simulink model "demoS175WindCurrentAutopilot"  (R2022a)
settings: Solver=ode45  StartTime=0.0  StopTime=500  FixedStep=Auto  RelTol=1e-10  EnableMultiTasking=on
PreLoadFcn:
  | TT=50;
InitFcn:
  | dataContainer;
StopFcn:
  | shipsOrient;
undefined symbols (not defined in the file): aH, AR, B, cpr, cpv, cRr, cRrrr, cRrrv, cRX, D, Delta, detM, epsilon, g, ga, GM, kk, Kp, Kphi, Kr, Krphiphi, Krrphi, Krrr, Kv, Kvphiphi, Kvrr, Kvvphi, Kvvr, Kvvv, L, lx, m, m11, m22, m32, m33, m42, m44, magnitude, mx, my, nabla, Np, Nphi, Nr, Nrphiphi, Nrrphi, Nrrr, Nv, Nvphiphi, Nvrr, Nvvphi, Nvvr, Nvvv, rho, tau, wp, xH, xp, Xphiphi ... (+18)
libraries: simulink_extras x8, mssSimulink x5, simulink x4
settings Model: Creator=AP  LastModifiedBy=thor
settings SolverCC: AlgebraicLoopSolver=TrustRegion
settings DataIOCC: LimitDataPoints=on  SaveFormat=Array  SignalLoggingSaveFormat=ModelDataLogs  ReturnWorkspaceOutputs=off
settings OptimizationCC: ExpressionDepthLimit=2147483647  InitFltsAndDblsToZero=on  LifeSpan=inf
settings DebuggingCC: SaveWithParameterizedLinksMsg=none  UnderspecifiedInitializationDetection=Classic  MergeDetectMultiDrivingBlocksExec=none  SignalResolutionControl=TryResolveAllWithWarning  SolverPrmCheckMsg=warning  MultiTaskDSMMsg=warning  MultiTaskCondExecSysMsg=none  FcnCallInpInsideContextMsg=warning  UnconnectedInputMsg=warning  UnconnectedOutputMsg=warning  UnconnectedLineMsg=warning  StateNameClashWarn=warning  SFUnexpectedBacktrackingDiag=warning  SFNoUnconditionalDefaultTransitionDiag=warning  SFExecutionAtInitializationDiag=none  SFMachineParentedDataDiag=warning  ArithmeticOperatorsInVariantConditions=warning
settings HardwareCC: ProdBitPerPointer=32  ProdBitPerSizeT=32  ProdBitPerPtrDiffT=32  ProdLargestAtomicFloat=None  ProdIntDivRoundTo=Undefined  ProdEndianess=Unspecified  ProdWordSize=32  ProdHWDeviceType=32-bit Generic
settings ModelReferenceCC: PropagateSignalLabelsOutOfModel=off
settings SFSimCC: SimUseLocalCustomCode=off  CustomCodeUndefinedFunction=UseInterfaceOnly
settings RTWCC: RTWUseLocalCustomCode=off  DLArmComputeVersion=19.05
settings CodeAppCC: StateflowObjectComments=on
settings GRTTargetCC: TargetFcnLib=ansi_tfl_tmw.mat  TargetLangStandard=C89/C90 (ANSI)  CombineOutputUpdateFcns=off  GRTInterface=on
settings ConfigComp: CovMetricSettings=dw  CovSaveCumulativeToWorkspaceVar=on  CovSaveSingleToWorkspaceVar=on  CovExternalEMLEnable=off

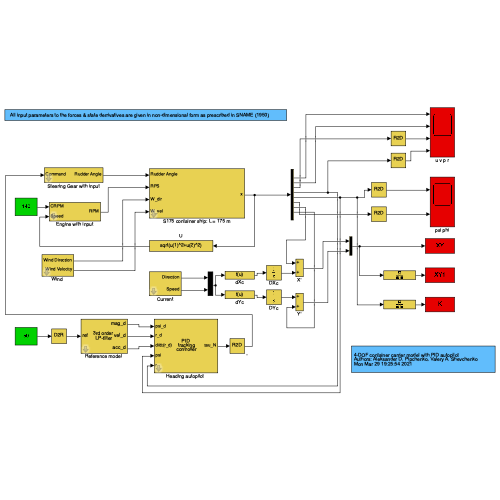
[thumbnail: Simulink's stored preview of the top-level diagram]
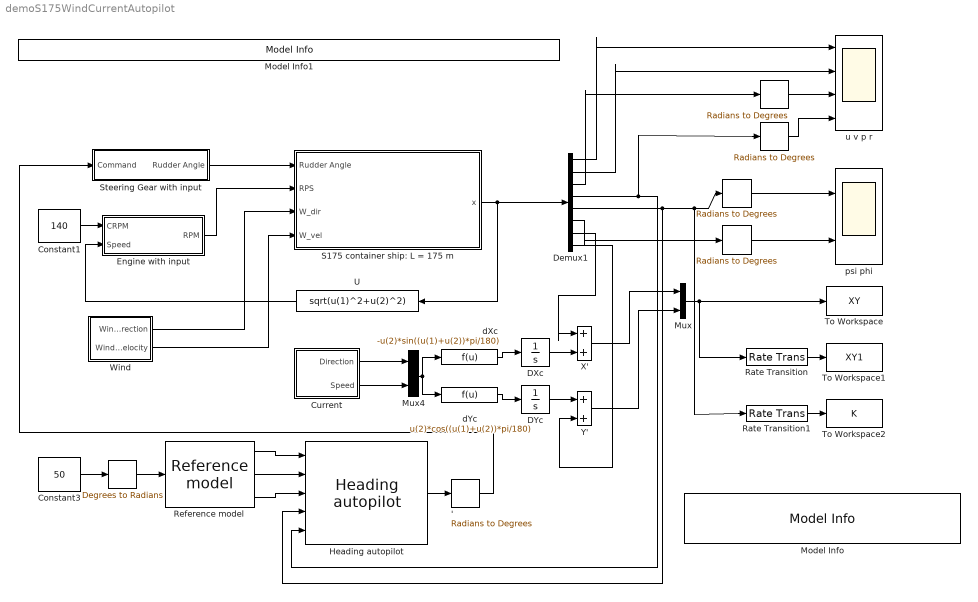
== system demoS175WindCurrentAutopilot ==
  "   " : simulink_extras/Transformations/Radians to Degrees
  "    " : simulink_extras/Transformations/Radians to Degrees
  "     " : simulink_extras/Transformations/Degrees to Radians
  "      " : simulink_extras/Transformations/Radians to Degrees
  "                " : simulink_extras/Transformations/Radians to Degrees
  "               '" : simulink_extras/Transformations/Radians to Degrees
  Constant1 : Constant  Value=140
  Constant3 : Constant  Value=50
  Current : Subsystem  AncestorBlock=Maneuvering/Environment/Current  mask(Environment disturbance/ Sea Current){CD=5, CS=2}
      mask prompts: CD "Current Direction, deg"; CS "Current Speed, knots"
      mask help: Apply current speed and direction to appropriate gaps
  DXc : Integrator
  DYc : Integrator
  Demux1 : Demux  Outputs=8
  Engine with input : Subsystem  mask(Engine (simplified)){IRPM=140, MaxRPM=160, MinRPM=0, T_rpm=5.65, RevV=0, RTH=0, OTE=Revs per second}
      mask prompts: IRPM "Initial RPM, revs/min"; MaxRPM "Maximum RPM"; MinRPM "Minimum RPM"; T_rpm "Derrivative Time Constant"; RevV "Reversal speed, m/s"; RTH "RPM to keep ahead at crash stop, revs/min"; OTE "Output time expression"
      mask help:
      | Insert the reversal speed, and RPM ahead you want to hold
      | while ship not reach this speed at crash stop maneuver
      mask init:
      | if OTE=='Revs per minute'
      | 	TEX = 1;
      | elseif OTE=='Revs per second'
      | 	TEX = 1/60;
      | end;
      mask TypeOptions OTE: Revs per minute | Revs per second
  "Heading autopilot " : mssSimulink/Control/Autopilots/Heading autopilot  T_nomoto=107.3  K_nomoto=0.185  Kp=2  Td=50  Ti=100
  Model Info : simulink/Model-Wide Utilities/Model Info  Frame=on  DisplayStringWithTags=|  HorizontalTextAlignment=Left  LeftAlignmentValue=0.02
      | 4-DOF container carrier model with PID autopilot
      | Authors: Aleksander D. Pipchenko, Valery A. Shevchenko
      | %<LastModificationDate>
  Model Info1 : simulink/Model-Wide Utilities/Model Info  Frame=on  DisplayStringWithTags=All input parameters to the forces & state derrivatives are given in non-dimensional form as prescribed in SNAME (1950)  HorizontalTextAlignment=Left  LeftAlignmentValue=0.02
  Mux : Mux  Inputs=2
  Mux4 : Mux  Inputs=2
  Rate Transition : RateTransition  OutPortSampleTime=TT
  Rate Transition1 : RateTransition  OutPortSampleTime=TT
  "Reference model " : mssSimulink/Guidance/Reference model  v_max=1.0  zeta_d=1.0  w_d=0.1
  S175 container ship: L = 175 m : Subsystem  mask(Container ship 4-DOF model / Simulink based){IC=[10 0.01 0 0 0 0 0 0]}
      mask prompts: IC "Initial conditions [u v p r psi phi X Y]"
      mask help:
      | Inputs/outputs:
      |
      |    Rudder Angle     - set in radians
      |    RPS              - propeller revolutions per second
      |    x                - state vector [u v p r psi phi X Y]
  Steering Gear with input : Subsystem  mask(Steering gear (simplified)){IRud=0, NSG=2, T_rud=1, DR=radians, MR=35, MRS=5, ST=-1}
      mask prompts: IRud "Intial Rudder angle, deg"; NSG "# of steering engnes in use"; T_rud "Derrivative time constant"; DR "Output values"; MR "Max. Rudder Angle, degrees"; MRS "Max. Rudder Speed, deg/second"; ST "Sample Time (-1 for inherited), s"
      mask init:
      | if DR=='degrees'
      | 	DRD = 1;
      | elseif DR=='radians'
      | 	DRD = pi/180;
      | end;
      mask TypeOptions NSG: 1 | 2
      mask TypeOptions DR: degrees | radians
  To Workspace : ToWorkspace  VariableName=XY  SampleTime=-1
  To Workspace1 : ToWorkspace  VariableName=XY1  SampleTime=TT
  To Workspace2 : ToWorkspace  VariableName=K  SampleTime=TT
  U : Fcn  Expr=sqrt(u(1)^2+u(2)^2)
  "Wind " : Subsystem  mask(Wind){page=1, Par_Wind_slowlyvar=on, Par_Wind_gust=on, Par_Wind_V=15, Par_Wind_angle=150, Par_Wind_spectrum_type=2, Par_Wind_z=20, Par_Wind_sample_time=1, Par_Wind_speed_T=10, Par_Wind_angle_T=10, Par_Wind_speed_noise_pow=1, Par_Wind_angle_noise_pow=0.01, Par_Wind_speed_rand_max=10, Par_Wind_angle_rand_max=pi/8, Par_Wind_speed_seed=5, Par_Wind_angle_seed=10, Par_Wind_phase_seed=1532, Par_Wind_kappa_H=0.0026, Par_Wind_L=1800, Par_Wind_minfreq=1E-4, Par_Wind_maxfreq=0.1, Par_Wind_nfreq=100}
      mask prompts: Par_Wind_slowlyvar "Include slowly-varing wind velocity and direction"; Par_Wind_gust "Include wind gust"; Par_Wind_V "Mean wind velocity [m/s]"; Par_Wind_angle "Mean wind angle [deg]"; Par_Wind_spectrum_type "Wind gust spectrum type"; Par_Wind_z "Height over water surface [m (for NORSOK wind spectrum)]"; Par_Wind_sample_time "Wind sample time [s]"; Par_Wind_speed_T "Wind speed time constant [s]"; Par_Wind_angle_T "Wind angle time constant [s]"; Par_Wind_speed_noise_pow "Wind speed noise power"; Par_Wind_angle_noise_pow "Wind angle noise power"; Par_Wind_speed_rand_max "Wind speed saturation [m/s] (max random variation about mean)"; Par_Wind_angle_rand_max "Wind angle saturation [rad] (max random variation about mean)"; Par_Wind_speed_seed "Wind speed random seed"; Par_Wind_angle_seed "Wind angle random seed"; Par_Wind_phase_seed "Wind gust phase seed"; Par_Wind_kappa_H "Sea surface drag coefficient for Harris wind spectrum (0.0026)"; Par_Wind_L "Scaling length for Harris wind spectrum (1800)"; Par_Wind_minfreq "Minimum frequency in gust [Hz] (1E-4)"; Par_Wind_maxfreq "Maximum frequency in gust [Hz] (0.1)"; Par_Wind_nfreq "Number of frequency components"
      mask help:
      | Generates wind speed and direction based on the mean angle and mean wind speed at 10 meters height. The total velocity is composed of a slowly-varying mean superposed with gusts based on a chosen wind spectrum. The direction is slowly-varying based on a random process.
      |
      | The wind spectrum types are:
      |
      | 1) Harris         (based on measurements over land)
      | 2) NORSOK   (based on measurements from the North Sea)
      mask Help:
      | <b>Part of the Marine Systems Simulator: MSS</b><p>Generate wind speed and direction based on the mean angle and mean wind
      | speed at 10 meters height. The total velocity is composed of a slowly-varying
      | mean superposed with gusts based on a chosen wind spectrum. The direction is
      | slowly-varying based on a random process.<br>
      | <br>
      | The wind spectrum types are:<br>
      | <br>
      | 1) Harris (based on measurements over land)<br>
      | 2) NORSOK (based on measurements from the North Sea)</p>
      | <p>The wind gust from the Harris spectrum is uniform over the height, whereas
      | the wind gust from the NORSOK spectrum varies with the height.</p>
      | <p>The random variation of the mean speed and angle can be limited by two saturation
      | parameters, which define the maximum random deviation from the mean value.<p><b>Outputs:
      | </b> </p>
      | <p>angle: [rad] Wind angle in the n-frame<br>
      | speed: [m/s] Wind velocity in the n-frame<p>
      | <b>Copyright NTNU 2005</b></p>
      | <p><b>Author:</b> Oyvind N. Smogeli, 2005-05-03</p>
      mask TypeOptions page: 1 | 2
      mask Callback page: MSS_mask_page(12);
      mask TypeOptions Par_Wind_spectrum_type: 1 | 2
  X' : Sum  SampleTime=1
  Y' : Sum  SampleTime=1
  dXc : Fcn  Expr=-u(2)*sin((u(1)+u(2))*pi/180)
  dYc : Fcn  Expr=u(2)*cos((u(1)+u(2))*pi/180)
  psi phi : Scope  NumInputPorts=2
  u v p r : Scope  NumInputPorts=4
  wires:
  "   "/1 -> psi phi/1
  Rate Transition/1 -> To Workspace1/1
  Rate Transition1/1 -> To Workspace2/1
  "    "/1 -> u v p r/3
  "      "/1 -> u v p r/4
  Steering Gear with input/1(Rudder Angle) -> S175 container ship: L = 175 m/1(Rudder Angle)
  S175 container ship: L = 175 m/1(x) -> U/1, Demux1/1
  Constant1/1 -> Engine with input/1(CRPM)
  U/1 -> Engine with input/2(Speed)
  "                "/1 -> psi phi/2
  Demux1/1 -> u v p r/1
  Demux1/2 -> u v p r/2
  Demux1/3 -> "    "/1
  Demux1/4 -> "      "/1, "Heading autopilot "/5
  Demux1/5 -> "   "/1, Rate Transition1/1, "Heading autopilot "/4
  Demux1/6 -> "                "/1
  Mux/1 -> To Workspace/1, Rate Transition/1
  "Wind "/1(Wind Direction) -> S175 container ship: L = 175 m/3(W_dir)
  Engine with input/1(RPM) -> S175 container ship: L = 175 m/2(RPS)
  "Wind "/2(Wind Velocity) -> S175 container ship: L = 175 m/4(W_vel)
  dXc/1 -> DXc/1
  dYc/1 -> DYc/1
  DXc/1 -> X'/2
  Current/1(Direction) -> Mux4/1
  Current/2(Speed) -> Mux4/2
  Mux4/1 -> dXc/1, dYc/1
  DYc/1 -> Y'/1
  X'/1 -> Mux/1
  Y'/1 -> Mux/2
  Demux1/7 -> X'/1
  Demux1/8 -> Y'/2
  "Reference model "/1 -> "Heading autopilot "/1
  "Reference model "/2 -> "Heading autopilot "/2
  "Reference model "/3 -> "Heading autopilot "/3
  "     "/1 -> "Reference model "/1
  Constant3/1 -> "     "/1
  "Heading autopilot "/1 -> "               '"/1
  "               '"/1 -> Steering Gear with input/1(Command)

== system demoS175WindCurrentAutopilot/Current ==
  Bias : Bias  Bias=-180  SaturateOnIntegerOverflow=off
  Bias1 : Bias  Bias=180  SaturateOnIntegerOverflow=off
  "Current Direction, deg" : Constant  Value=CD
  "Current Speed, knots" : Constant  Value=CS
  Gain : Gain  Gain=1853/3600
  Switch : Switch  Threshold=180  SaturateOnIntegerOverflow=off  InputSameDT=off
  Direction : Outport
  Speed : Outport  Port=2
  wires:
  Bias1/1 -> Switch/3
  Bias/1 -> Switch/1
  "Current Direction, deg"/1 -> Bias1/1, Bias/1, Switch/2
  Switch/1 -> Direction/1
  "Current Speed, knots"/1 -> Gain/1
  Gain/1 -> Speed/1

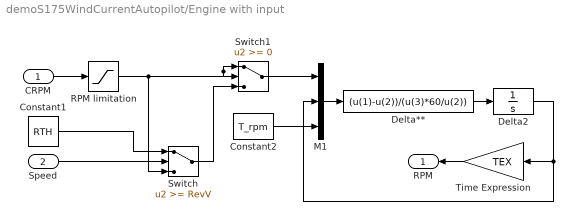
== system demoS175WindCurrentAutopilot/Engine with input ==
  CRPM : Inport
  Speed : Inport  Port=2
  Constant1 : Constant  Value=RTH
  Constant2 : Constant  Value=T_rpm
  Delta** : Fcn  Expr=(u(1)-u(2))/(u(3)*60/u(2))
  Delta2 : Integrator  InitialCondition=IRPM  LimitOutput=on  UpperSaturationLimit=MaxRPM  LowerSaturationLimit=MinRPM
  M1 : Mux  Inputs=3
  RPM limitation : Saturate  UpperLimit=MaxRPM  LowerLimit=MinRPM
  Switch : Switch  Threshold=RevV  SaturateOnIntegerOverflow=off  InputSameDT=off
  Switch1 : Switch  SaturateOnIntegerOverflow=off  InputSameDT=off
  Time Expression : Gain  Gain=TEX
  RPM : Outport
  wires:
  Constant2/1 -> M1/3
  RPM limitation/1 -> Switch1/1, Switch1/2, Switch/3
  CRPM/1 -> RPM limitation/1
  Switch/1 -> Switch1/3
  Speed/1 -> Switch/2
  Switch1/1 -> M1/1
  Constant1/1 -> Switch/1
  M1/1 -> Delta**/1
  Delta**/1 -> Delta2/1
  Delta2/1 -> M1/2, Time Expression/1
  Time Expression/1 -> RPM/1

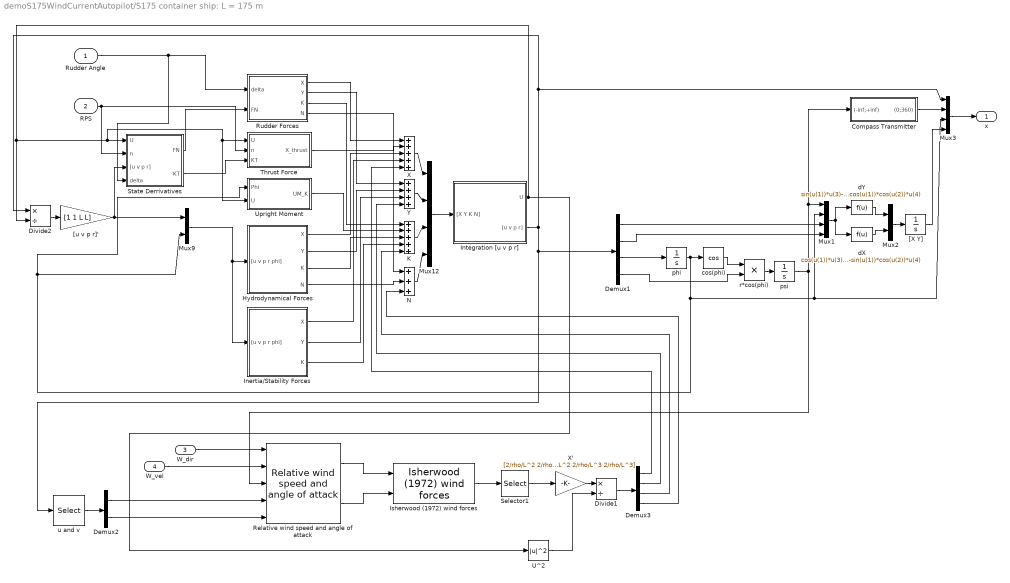
== system demoS175WindCurrentAutopilot/S175 container ship: L = 175 m ==
  Rudder Angle : Inport
  RPS : Inport  Port=2
  W_dir : Inport  Port=3
  W_vel : Inport  Port=4
  Compass Transmitter : Subsystem  mask(Compass Transmitter){IVS=radians, OVS=radians}
      mask prompts: IVS "Input Value"; OVS "Output Value"
      mask help:
      | This block transfers the input value ranged (-inf;+inf) to value ranged (0;360) or (0;2*pi)
      | according to your choice.
      mask init:
      | if IVS =='degrees' 
      | 	IV =1;
      | elseif IVS =='radians'
      | 	IV = 180/pi;
      | end;
      | if OVS =='degrees'
      | 	OV =1;
      | elseif OVS=='radians'
      | 	OV=pi/180;
      | end;
      mask TypeOptions IVS: degrees | radians
      mask TypeOptions OVS: degrees | radians
  Demux1 : Demux
  Demux2 : Demux  Outputs=2
  Demux3 : Demux
  Divide1 : Product  Inputs=*/
  Divide2 : Product  Inputs=*/
  Hydrodynamical Forces : Subsystem
  Inertia/Stability Forces : Subsystem
  Integration [u v p r] : Subsystem
  "Isherwood (1972) wind forces  " : mssSimulink/Environment/Wind/Isherwood (1972) wind forces  L=L  B=B  A_T=100  A_L=2000  A_SS=200  S=130  C=30  M=0
  K : Sum  Inputs=+++++
  Mux1 : Mux
  Mux12 : Mux
  Mux2 : Mux  Inputs=2
  Mux3 : Mux
  Mux9 : Mux  Inputs=2
  N : Sum  Inputs=+++
  "Relative wind speed and angle of attack " : mssSimulink/Environment/Wind/Relative wind speed and angle of attack  SystemSampleTime=-1  VariantActivationTime=update diagram  Latency=0  AutoFrameSizeCalculation=off
  Rudder Forces : Subsystem
  Selector1 : Selector  InputPortWidth=6  IndexOptions=Index vector (dialog)  Indices=[1 2 4 6]  OutputSizes=1
  State Derrivatives : Subsystem
  Thrust Force : Subsystem
  U^2 : Math  Operator=magnitude^2  SignedPower=on
  Upright Moment : Subsystem
  X : Sum  Inputs=+++++
  X' : Gain  Gain=[2/rho/L^2 2/rho/L^2 2/rho/L^3 2/rho/L^3]
  Y : Sum  Inputs=++++
  "[X Y]" : Integrator  InitialCondition=[IC(7) IC(8)]
  "[u v p r]'" : Gain  Gain=[1 1 L L]
  cos(phi) : Trigonometry  Operator=cos
  dX : Fcn  Expr=cos(u(1))*u(3)-sin(u(1))*cos(u(2))*u(4)
  dY : Fcn  Expr=sin(u(1))*u(3)-cos(u(1))*cos(u(2))*u(4)
  phi : Integrator  InitialCondition=IC(6)
  psi : Integrator  InitialCondition=IC(5)
  r*cos(phi) : Product  Inputs=**
  u and v : Selector  InputPortWidth=4  IndexOptions=Index vector (dialog)  Indices=[1 2]  OutputSizes=1
  x : Outport
  wires:
  "[u v p r]'"/1 -> Mux9/1, State Derrivatives/3("[u v p r]")
  Divide2/1 -> "[u v p r]'"/1
  X/1 -> Mux12/1
  Y/1 -> Mux12/2
  K/1 -> Mux12/3
  N/1 -> Mux12/4
  Integration [u v p r]/2("[u v p r]") -> Divide2/1, Mux3/1, Demux1/1, u and v/1
  Mux12/1 -> Integration [u v p r]/1("[X Y K N]")
  Integration [u v p r]/1(U) -> Divide2/2, Thrust Force/1(U), Upright Moment/2(U), State Derrivatives/1(U), U^2/1
  State Derrivatives/1(FN) -> Rudder Forces/2(FN)
  State Derrivatives/2(KT) -> Thrust Force/3(KT)
  Rudder Angle/1 -> Rudder Forces/1(delta), State Derrivatives/4(delta)
  Mux9/1 -> Hydrodynamical Forces/1("[u v p r phi]"), Inertia/Stability Forces/1("[u v p r phi]")
  Rudder Forces/1(X) -> X/1
  Thrust Force/1(X_thrust) -> X/2
  Hydrodynamical Forces/1(X) -> X/3
  Inertia/Stability Forces/1(X) -> X/4
  Rudder Forces/2(Y) -> Y/1
  Hydrodynamical Forces/2(Y) -> Y/2
  Inertia/Stability Forces/2(Y) -> Y/3
  Rudder Forces/3(K) -> K/1
  Upright Moment/1(UM_K) -> K/2
  Hydrodynamical Forces/3(K) -> K/3
  Inertia/Stability Forces/3(K) -> K/4
  Hydrodynamical Forces/4(N) -> N/2
  Rudder Forces/4(N) -> N/1
  RPS/1 -> Thrust Force/2(n), State Derrivatives/2(n)
  Demux1/1 -> Mux1/3
  Demux1/2 -> Mux1/4
  Demux1/3 -> phi/1
  Demux1/4 -> r*cos(phi)/2
  phi/1 -> Upright Moment/1(Phi), Mux9/2, Mux1/2, Mux3/3, cos(phi)/1
  cos(phi)/1 -> r*cos(phi)/1
  r*cos(phi)/1 -> psi/1
  psi/1 -> "Relative wind speed and angle of attack "/3, Mux1/1, Compass Transmitter/1((-inf;+inf))
  Mux1/1 -> dX/1, dY/1
  dY/1 -> Mux2/1
  dX/1 -> Mux2/2
  Mux2/1 -> "[X Y]"/1
  Mux3/1 -> x/1
  Compass Transmitter/1((0;360)) -> Mux3/2
  "[X Y]"/1 -> Mux3/4
  "Relative wind speed and angle of attack "/2 -> "Isherwood (1972) wind forces  "/2
  Demux2/2 -> "Relative wind speed and angle of attack "/5
  Demux2/1 -> "Relative wind speed and angle of attack "/4
  "Isherwood (1972) wind forces  "/1 -> Selector1/1
  U^2/1 -> Divide1/2
  X'/1 -> Divide1/1
  Selector1/1 -> X'/1
  Divide1/1 -> Demux3/1
  u and v/1 -> Demux2/1
  "Relative wind speed and angle of attack "/1 -> "Isherwood (1972) wind forces  "/1
  W_dir/1 -> "Relative wind speed and angle of attack "/1
  W_vel/1 -> "Relative wind speed and angle of attack "/2
  Demux3/1 -> X/5
  Demux3/2 -> Y/4
  Demux3/3 -> K/5
  Demux3/4 -> N/3

== system demoS175WindCurrentAutopilot/Steering Gear with input ==
  note: Steering Gears/Time constant
  Command : Inport
  Constant1 : Constant  Value=NSG/T_rud
  Delta : Integrator  InitialCondition=IRud  LimitOutput=on  UpperSaturationLimit=MR  LowerSaturationLimit=-MR
  Delta* : Fcn  Expr=u(2)*(u(1)-u(3))  SampleTime=ST
  M1 : Mux  Inputs=3
  RDL : Saturate  UpperLimit=MRS  LowerLimit=-MRS  SampleTime=ST
  Rudder limitation : Saturate  UpperLimit=MR  LowerLimit=-MR  SampleTime=ST
  angle transform : Gain  Gain=DRD  SampleTime=ST
  Rudder Angle : Outport
  wires:
  RDL/1 -> Delta/1
  angle transform/1 -> Rudder Angle/1
  Constant1/1 -> M1/2
  Rudder limitation/1 -> M1/1
  Delta/1 -> M1/3, angle transform/1
  Delta*/1 -> RDL/1
  M1/1 -> Delta*/1
  Command/1 -> Rudder limitation/1

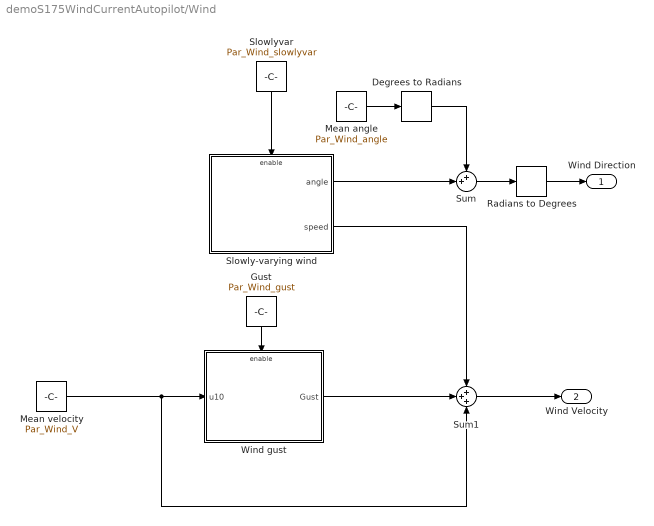
== system demoS175WindCurrentAutopilot/Wind  ==
  Degrees to Radians : simulink_extras/Transformations/Degrees to Radians
  Gust : Constant  Value=Par_Wind_gust
  Mean angle : Constant  Value=Par_Wind_angle
  Mean velocity : Constant  Value=Par_Wind_V
  Radians to Degrees : simulink_extras/Transformations/Radians to Degrees
  Slowly-varying wind : Subsystem  mask(Slowly-varying wind){Par_Wind_sample_time=Par_Wind_sample_time, Par_Wind_speed_T=Par_Wind_speed_T, Par_Wind_angle_T=Par_Wind_angle_T, Par_Wind_speed_noise_pow=Par_Wind_speed_noise_pow, Par_Wind_angle_noise_pow=Par_Wind_angle_noise_pow, Par_Wind_speed_rand_max=Par_Wind_speed_rand_max, Par_Wind_angle_rand_max=Par_Wind_angle_rand_max, Par_Wind_speed_seed=Par_Wind_speed_seed, Par_Wind_angle_seed=Par_Wind_angle_seed}
      mask prompts: Par_Wind_sample_time "Wind sample time [s]"; Par_Wind_speed_T "Wind speed time constant [s]"; Par_Wind_angle_T "Wind angle time constant [s]"; Par_Wind_speed_noise_pow "Wind speed noise power"; Par_Wind_angle_noise_pow "Wind angle noise power"; Par_Wind_speed_rand_max "Wind speed saturation [m/s] (max random variation about mean)"; Par_Wind_angle_rand_max "Wind angle saturation [rad] (max random variation about mean)"; Par_Wind_speed_seed "Wind speed random seed"; Par_Wind_angle_seed "Wind angle random seed"
      mask help:
      | Generate slowly varying wind speed and direction based on random processes.
      |
      | stochastic = 0  gives constant mean wind speed and direction
      | stochastic = 1  gives stochastic mean wind speed and direction
      mask Help:
      | Generate slowly varying wind speed and direction based on random processes.<br>
      | <br>
      | stochastic = 0 gives constant mean wind direction and speed,<br>
      | stochastic = 1 gives stochastic mean wind direction and speed<br>
      | <br>
      | <p>The randomness of the mean speed and angle can be limited by two saturation
      | parameters, which define the maximum random deviation from the mean value.<br>
  Slowlyvar : Constant  Value=Par_Wind_slowlyvar
  Sum : Sum  Inputs=++|  SaturateOnIntegerOverflow=on
  Sum1 : Sum  Inputs=+++  SaturateOnIntegerOverflow=on
  Wind gust : Subsystem  mask(Wind gust){Par_Wind_spectrum_type=Par_Wind_spectrum_type, Par_Wind_phase_seed=Par_Wind_phase_seed, Par_Wind_kappa_H=Par_Wind_kappa_H, Par_Wind_L=Par_Wind_L, Par_Wind_z=Par_Wind_z, Par_Wind_minfreq=Par_Wind_minfreq, Par_Wind_maxfreq=Par_Wind_maxfreq, Par_Wind_nfreq=Par_Wind_nfreq}
      mask prompts: Par_Wind_spectrum_type "Spectrum type"; Par_Wind_phase_seed "Wind gust phase seed"; Par_Wind_kappa_H "Sea surface drag coefficient for Harris wind spectrum (0.0026)"; Par_Wind_L "Scaling length for Harris wind spectrum (1800)"; Par_Wind_z "Height over water surface, for NORSOK spectrum"; Par_Wind_minfreq "Minimum frequency in gust [Hz] (1E-4)"; Par_Wind_maxfreq "Maximum frequency in gust [Hz] (0.1)"; Par_Wind_nfreq "Number of frequency components"
      mask help:
      | Calculate the wind gust according to one of two gust spectra:
      |
      | 1) Harris (based on measurements over land)
      | 2) NORSOK (based on measurements from the North Sea)
      |
      | The gust from the Harris spectrum is not influenced by the heigth over the sea surface, whereas the gust from the NORSOK spectrum is.
  Wind Direction : Outport
  Wind Velocity : Outport  Port=2
  wires:
  Degrees to Radians/1 -> Sum/1
  Radians to Degrees/1 -> Wind Direction/1
  Gust/1 -> Wind gust/Enable
  Slowlyvar/1 -> Slowly-varying wind/Enable
  Slowly-varying wind/1(angle) -> Sum/2
  Mean velocity/1 -> Wind gust/1(u10), Sum1/3
  Mean angle/1 -> Degrees to Radians/1
  Sum/1 -> Radians to Degrees/1
  Wind gust/1(Gust) -> Sum1/2
  Slowly-varying wind/2(speed) -> Sum1/1
  Sum1/1 -> Wind Velocity/1

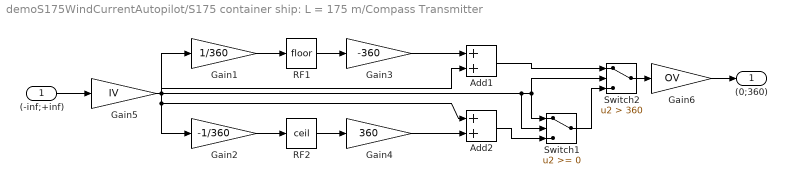
== system demoS175WindCurrentAutopilot/S175 container ship: L = 175 m/Compass Transmitter ==
  (-inf;+inf) : Inport
  Add1 : Sum
  Add2 : Sum
  Gain1 : Gain  Gain=1/360
  Gain2 : Gain  Gain=-1/360
  Gain3 : Gain  Gain=-360
  Gain4 : Gain  Gain=360
  Gain5 : Gain  Gain=IV
  Gain6 : Gain  Gain=OV
  RF1 : Rounding
  RF2 : Rounding  Operator=ceil
  Switch1 : Switch  SaturateOnIntegerOverflow=off  InputSameDT=off
  Switch2 : Switch  Criteria=u2 > Threshold  Threshold=360  SaturateOnIntegerOverflow=off  InputSameDT=off
  (0;360) : Outport
  wires:
  Gain6/1 -> (0;360)/1
  Gain5/1 -> Switch1/2, Switch2/2, Switch1/1, Gain1/1, Add1/2, Gain2/1, Add2/1
  Switch2/1 -> Gain6/1
  Switch1/1 -> Switch2/3
  Add2/1 -> Switch1/3
  Add1/1 -> Switch2/1
  Gain4/1 -> Add2/2
  Gain3/1 -> Add1/1
  RF2/1 -> Gain4/1
  RF1/1 -> Gain3/1
  Gain2/1 -> RF2/1
  Gain1/1 -> RF1/1
  (-inf;+inf)/1 -> Gain5/1

== system demoS175WindCurrentAutopilot/S175 container ship: L = 175 m/Hydrodynamical Forces ==
  "[u v p r phi]" : Inport
  Khydro : Fcn  Expr=Kv*u(2) + Kr*u(4) + Kp*u(3) + Kphi*u(5) + Kvvv*u(2)^3 + Krrr*u(4)^3 + Kvvr*u(2)^2*u(4) + Kvrr*u(2)*u(4)^2 + Kvvphi*u(2)^2*u(5) + Kvphiphi*u(2)*u(5)^2 + Krrphi*u(4)^2*u(5) + Krphiphi*u(4)*u(5)^2
  Nhydro : Fcn  Expr=Nv*u(2) + Nr*u(4) + Np*u(3) + Nphi*u(5) + Nvvv*u(2)^3 + Nrrr*u(4)^3 + Nvvr*u(2)^2*u(4) + Nvrr*u(2)*u(4)^2 + Nvvphi*u(2)^2*u(5) + Nvphiphi*u(2)*u(5)^2 + Nrrphi*u(4)^2*u(5) + Nrphiphi*u(4)*u(5)^2
  Xhydro : Fcn  Expr="Xuu*u(1)^2 +  Xvr*u(2)*u(4) + Xvv*u(2)^2 + Xrr*u(4)^2 + Xphiphi*u(5)^2"
  Yhydro : Fcn  Expr=Yv*u(2) + Yr*u(4) + Yp*u(3) + Yphi*u(5) + Yvvv*u(2)^3 + Yrrr*u(4)^3 + Yvvr*u(2)^2*u(4) + Yvrr*u(2)*u(4)^2 + Yvvphi*u(2)^2*u(5) + Yvphiphi*u(2)*u(5)^2 + Yrrphi*u(4)^2*u(5) + Yrphiphi*u(4)*u(5)^2
  X : Outport
  Y : Outport  Port=2
  K : Outport  Port=3
  N : Outport  Port=4
  wires:
  "[u v p r phi]"/1 -> Xhydro/1, Yhydro/1, Khydro/1, Nhydro/1
  Xhydro/1 -> X/1
  Yhydro/1 -> Y/1
  Khydro/1 -> K/1
  Nhydro/1 -> N/1

== system demoS175WindCurrentAutopilot/S175 container ship: L = 175 m/Inertia//Stability Forces ==
  "[u v p r phi]" : Inport
  Kinertia : Fcn  Expr=mx*lx*u(1)*u(4)
  Xinertia : Fcn  Expr=(m + my)*u(2)*u(4)
  Yinertia : Fcn  Expr=- (m + mx)*u(1)*u(4)
  X : Outport
  Y : Outport  Port=2
  K : Outport  Port=3
  wires:
  "[u v p r phi]"/1 -> Xinertia/1, Yinertia/1, Kinertia/1
  Xinertia/1 -> X/1
  Yinertia/1 -> Y/1
  Kinertia/1 -> K/1

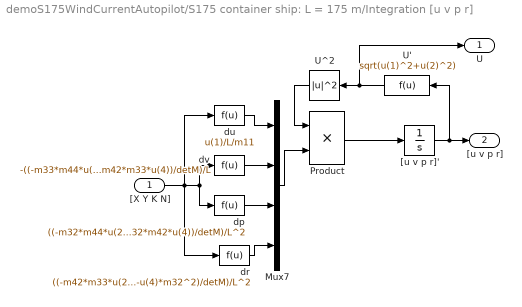
== system demoS175WindCurrentAutopilot/S175 container ship: L = 175 m/Integration [u v p r] ==
  "[X Y K N]" : Inport
  Mux7 : Mux
  Product : Product  Inputs=**
  U' : Fcn  Expr=sqrt(u(1)^2+u(2)^2)
  U^2 : Math  Operator=magnitude^2  SignedPower=on
  "[u v p r]'" : Integrator  InitialCondition=[IC(1:4)]
  dp : Fcn  Expr=((-m32*m44*u(2)+u(3)*m22*m44-u(3)*m42^2+m32*m42*u(4))/detM)/L^2
  dr : Fcn  Expr=((-m42*m33*u(2)+m32*m42*u(3)+u(4)*m22*m33-u(4)*m32^2)/detM)/L^2
  du : Fcn  Expr=u(1)/L/m11
  dv : Fcn  Expr=-((-m33*m44*u(2)+m32*m44*u(3)+m42*m33*u(4))/detM)/L
  U : Outport
  "[u v p r]" : Outport  Port=2
  wires:
  du/1 -> Mux7/1
  dv/1 -> Mux7/2
  dp/1 -> Mux7/3
  dr/1 -> Mux7/4
  Mux7/1 -> Product/2
  U^2/1 -> Product/1
  "[u v p r]'"/1 -> "[u v p r]"/1, U'/1
  Product/1 -> "[u v p r]'"/1
  "[X Y K N]"/1 -> dp/1, dv/1, dr/1, du/1
  U'/1 -> U^2/1, U/1

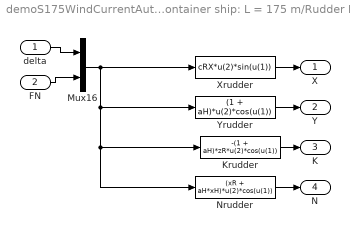
== system demoS175WindCurrentAutopilot/S175 container ship: L = 175 m/Rudder Forces ==
  delta : Inport
  FN : Inport  Port=2
  Krudder : Fcn  Expr=-(1 + aH)*zR*u(2)*cos(u(1))
  Mux16 : Mux  Inputs=2
  Nrudder : Fcn  Expr=(xR + aH*xH)*u(2)*cos(u(1))
  Xrudder : Fcn  Expr=cRX*u(2)*sin(u(1))
  Yrudder : Fcn  Expr=(1 + aH)*u(2)*cos(u(1))
  X : Outport
  Y : Outport  Port=2
  K : Outport  Port=3
  N : Outport  Port=4
  wires:
  Mux16/1 -> Xrudder/1, Yrudder/1, Krudder/1, Nrudder/1
  Xrudder/1 -> X/1
  Yrudder/1 -> Y/1
  Krudder/1 -> K/1
  Nrudder/1 -> N/1
  delta/1 -> Mux16/1
  FN/1 -> Mux16/2

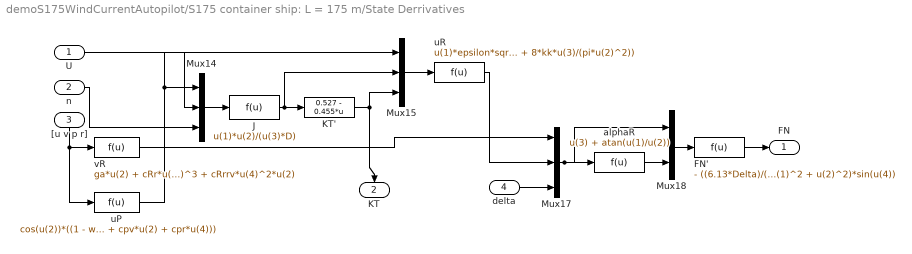
== system demoS175WindCurrentAutopilot/S175 container ship: L = 175 m/State Derrivatives ==
  U : Inport
  n : Inport  Port=2
  "[u v p r]" : Inport  Port=3
  delta : Inport  Port=4
  FN' : Fcn  Expr=- ((6.13*Delta)/(Delta + 2.25))*(AR/L^2)*(u(1)^2 + u(2)^2)*sin(u(4))
  J : Fcn  Expr=u(1)*u(2)/(u(3)*D)
  KT' : Fcn  Expr=0.527 - 0.455*u
  Mux14 : Mux  Inputs=3
  Mux15 : Mux  Inputs=3
  Mux17 : Mux  Inputs=3
  Mux18 : Mux  Inputs=2
  alphaR : Fcn  Expr=u(3) + atan(u(1)/u(2))
  uP : Fcn  Expr=cos(u(2))*((1 - wp) + tau*((u(2) + xp*u(4))^2 + cpv*u(2) + cpr*u(4)))
  uR : Fcn  Expr=u(1)*epsilon*sqrt(1 + 8*kk*u(3)/(pi*u(2)^2))
  vR : Fcn  Expr=ga*u(2) + cRr*u(4) + cRrrr*u(4)^3 + cRrrv*u(4)^2*u(2)
  FN : Outport
  KT : Outport  Port=2
  wires:
  alphaR/1 -> Mux18/2
  Mux18/1 -> FN'/1
  vR/1 -> Mux17/1
  Mux17/1 -> alphaR/1, Mux18/1
  uR/1 -> Mux17/2
  KT'/1 -> Mux15/3, KT/1
  Mux15/1 -> uR/1
  uP/1 -> Mux14/1, Mux15/1
  J/1 -> KT'/1, Mux15/2
  Mux14/1 -> J/1
  U/1 -> Mux14/2
  n/1 -> Mux14/3
  "[u v p r]"/1 -> vR/1, uP/1
  delta/1 -> Mux17/3
  FN'/1 -> FN/1

== system demoS175WindCurrentAutopilot/S175 container ship: L = 175 m/Thrust Force ==
  U : Inport
  n : Inport  Port=2
  KT : Inport  Port=3
  Mux19 : Mux  Inputs=3
  T : Fcn  Expr=2*rho*D^4/(u(1)^2*L^2*rho)*u(3)*u(2)*abs(u(2))
  Xthrust : Gain  Gain=1-t
  X_thrust : Outport
  wires:
  Mux19/1 -> T/1
  T/1 -> Xthrust/1
  U/1 -> Mux19/1
  n/1 -> Mux19/2
  Xthrust/1 -> X_thrust/1
  KT/1 -> Mux19/3

== system demoS175WindCurrentAutopilot/S175 container ship: L = 175 m/Upright Moment ==
  Phi : Inport
  U : Inport  Port=2
  Divide1 : Product  Inputs=**
  K_upright_moment : Gain  Gain=-GM
  W : Fcn  Expr=rho*g*nabla/(rho*L^2*u^2/2)
  UM_K : Outport
  wires:
  W/1 -> Divide1/2
  Divide1/1 -> K_upright_moment/1
  Phi/1 -> Divide1/1
  U/1 -> W/1
  K_upright_moment/1 -> UM_K/1

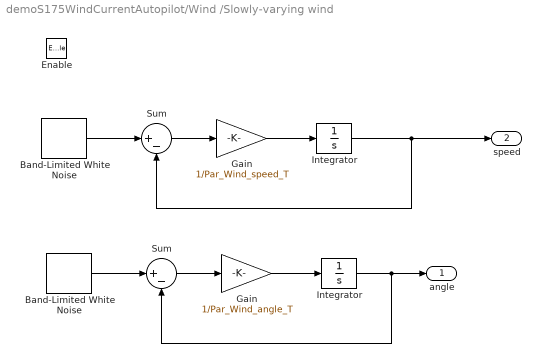
== system demoS175WindCurrentAutopilot/Wind /Slowly-varying wind ==
  Enable : EnablePort
  Band-Limited White Noise : simulink/Sources/Band-Limited White Noise  Cov=Par_Wind_speed_noise_pow  Ts=Par_Wind_sample_time  seed=Par_Wind_speed_seed
  "Band-Limited White Noise " : simulink/Sources/Band-Limited White Noise  Cov=Par_Wind_angle_noise_pow  Ts=Par_Wind_sample_time  seed=Par_Wind_angle_seed
  Gain : Gain  Gain=1/Par_Wind_speed_T  SaturateOnIntegerOverflow=on  OutDataTypeStr=Inherit: Same as input  ParamDataTypeStr=Inherit: Same as input
  "Gain " : Gain  Gain=1/Par_Wind_angle_T  SaturateOnIntegerOverflow=on  OutDataTypeStr=Inherit: Same as input  ParamDataTypeStr=Inherit: Same as input
  Integrator : Integrator  LimitOutput=on  UpperSaturationLimit=Par_Wind_speed_rand_max  LowerSaturationLimit=-Par_Wind_speed_rand_max
  "Integrator " : Integrator  LimitOutput=on  UpperSaturationLimit=Par_Wind_angle_rand_max  LowerSaturationLimit=-Par_Wind_angle_rand_max
  Sum : Sum  Inputs=|+-  InputSameDT=on  SaturateOnIntegerOverflow=on  OutDataTypeStr=Inherit: Same as first input
  "Sum       " : Sum  Inputs=|+-  InputSameDT=on  SaturateOnIntegerOverflow=on  OutDataTypeStr=Inherit: Same as first input
  angle : Outport  InitialOutput=0
  speed : Outport  Port=2  InitialOutput=0
  wires:
  Band-Limited White Noise/1 -> Sum/1
  Integrator/1 -> Sum/2, speed/1
  Sum/1 -> Gain/1
  Gain/1 -> Integrator/1
  "Band-Limited White Noise "/1 -> "Sum       "/1
  "Integrator "/1 -> "Sum       "/2, angle/1
  "Sum       "/1 -> "Gain "/1
  "Gain "/1 -> "Integrator "/1

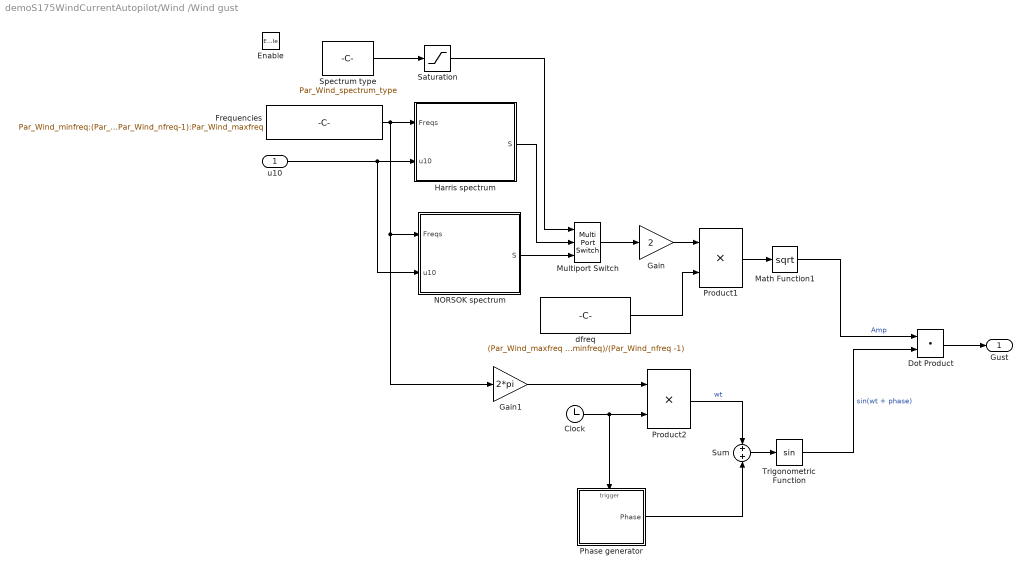
== system demoS175WindCurrentAutopilot/Wind /Wind gust ==
  u10 : Inport
  Enable : EnablePort
  Clock : Clock
  Dot Product : DotProduct  OutDataTypeStr=Inherit: Inherit via internal rule
  Frequencies : Constant  Value=Par_Wind_minfreq:(Par_Wind_maxfreq - Par_Wind_minfreq)/(Par_Wind_nfreq-1):Par_Wind_maxfreq
  Gain : Gain  Gain=2  SaturateOnIntegerOverflow=on  OutDataTypeStr=Inherit: Same as input  ParamDataTypeStr=Inherit: Same as input
  Gain1 : Gain  Gain=2*pi  SaturateOnIntegerOverflow=on  OutDataTypeStr=Inherit: Same as input  ParamDataTypeStr=Inherit: Same as input
  Harris spectrum : Subsystem
  Math Function1 : Math  Operator=sqrt  SignedPower=on
  Multiport Switch : MultiPortSwitch  Inputs=2  RndMeth=Nearest  InputSameDT=off
  NORSOK spectrum : Subsystem
  Phase generator : Subsystem
  Product1 : Product  SaturateOnIntegerOverflow=on  OutDataTypeStr=Inherit: Same as first input
  Product2 : Product  SaturateOnIntegerOverflow=on  OutDataTypeStr=Inherit: Same as first input
  Saturation : Saturate  UpperLimit=2  LowerLimit=1
  Spectrum type : Constant  Value=Par_Wind_spectrum_type
  Sum : Sum  SaturateOnIntegerOverflow=on
  Trigonometric Function : Trigonometry
  dfreq : Constant  Value=(Par_Wind_maxfreq - Par_Wind_minfreq)/(Par_Wind_nfreq -1)
  Gust : Outport  InitialOutput=0
  wires:
  Saturation/1 -> Multiport Switch/1
  Frequencies/1 -> Harris spectrum/1(Freqs), NORSOK spectrum/1(Freqs), Gain1/1
  u10/1 -> NORSOK spectrum/2(u10), Harris spectrum/2(u10)
  Gain/1 -> Product1/1
  dfreq/1 -> Product1/2
  Product1/1 -> Math Function1/1
  Multiport Switch/1 -> Gain/1
  Spectrum type/1 -> Saturation/1
  Harris spectrum/1(S) -> Multiport Switch/2
  NORSOK spectrum/1(S) -> Multiport Switch/3
  Gain1/1 -> Product2/1
  Clock/1 -> Product2/2, Phase generator/Trigger
  Product2/1 -> Sum/1  "wt"
  Phase generator/1(Phase) -> Sum/2
  Sum/1 -> Trigonometric Function/1
  Math Function1/1 -> Dot Product/1  "Amp"
  Trigonometric Function/1 -> Dot Product/2  "sin(wt + phase)"
  Dot Product/1 -> Gust/1

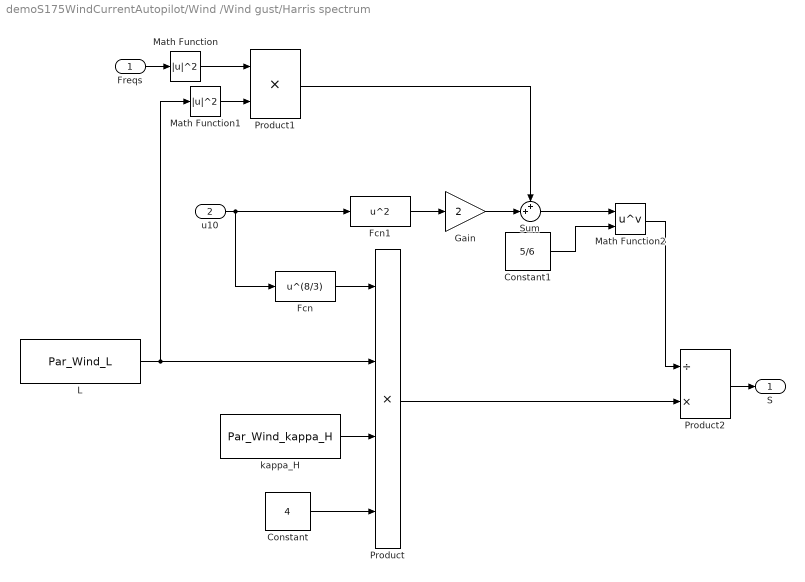
== system demoS175WindCurrentAutopilot/Wind /Wind gust/Harris spectrum ==
  Freqs : Inport
  u10 : Inport  Port=2
  Constant : Constant  Value=4
  Constant1 : Constant  Value=5/6
  Fcn : Fcn  Expr=u^(8/3)
  Fcn1 : Fcn  Expr=u^2
  Gain : Gain  Gain=2  SaturateOnIntegerOverflow=on  OutDataTypeStr=Inherit: Same as input  ParamDataTypeStr=Inherit: Same as input
  L : Constant  Value=Par_Wind_L
  Math Function : Math  Operator=magnitude^2  SignedPower=on
  Math Function1 : Math  Operator=magnitude^2  SignedPower=on
  Math Function2 : Math  Operator=pow  SignedPower=on
  Product : Product  Inputs=4  SaturateOnIntegerOverflow=on  OutDataTypeStr=Inherit: Same as first input
  Product1 : Product  SaturateOnIntegerOverflow=on  OutDataTypeStr=Inherit: Same as first input
  Product2 : Product  Inputs=/*  SaturateOnIntegerOverflow=on  OutDataTypeStr=Inherit: Same as first input
  Sum : Sum  Inputs=++|  SaturateOnIntegerOverflow=on
  kappa_H : Constant  Value=Par_Wind_kappa_H
  S : Outport
  wires:
  kappa_H/1 -> Product/3
  Fcn/1 -> Product/1
  u10/1 -> Fcn1/1, Fcn/1
  Fcn1/1 -> Gain/1
  Gain/1 -> Sum/2
  Constant/1 -> Product/4
  L/1 -> Product/2, Math Function1/1
  Math Function/1 -> Product1/1
  Math Function1/1 -> Product1/2
  Product1/1 -> Sum/1
  Sum/1 -> Math Function2/1
  Constant1/1 -> Math Function2/2
  Math Function2/1 -> Product2/1
  Product/1 -> Product2/2
  Freqs/1 -> Math Function/1
  Product2/1 -> S/1

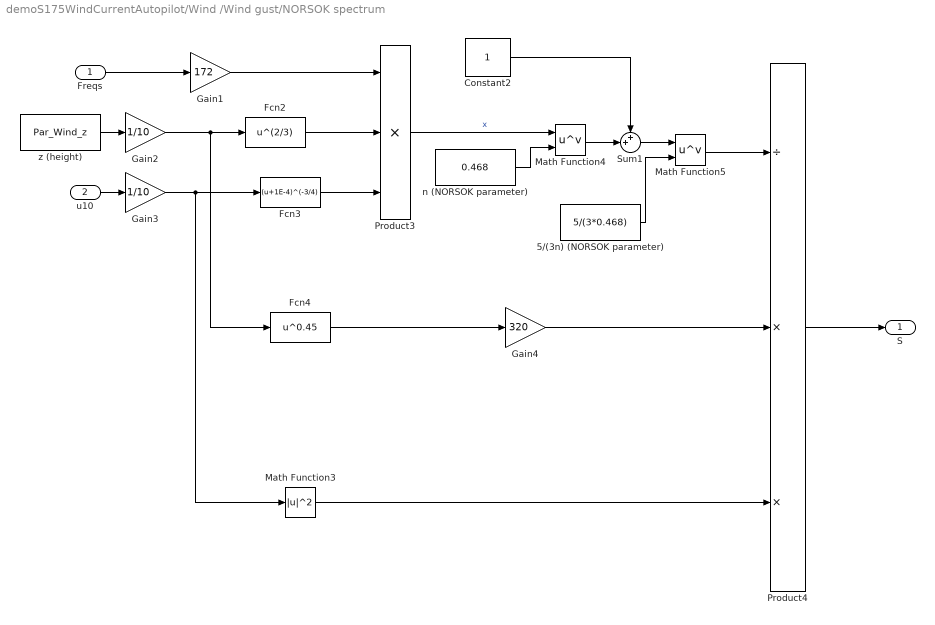
== system demoS175WindCurrentAutopilot/Wind /Wind gust/NORSOK spectrum ==
  Freqs : Inport
  u10 : Inport  Port=2
  5/(3n) (NORSOK parameter) : Constant  Value=5/(3*0.468)
  Constant2 : Constant
  Fcn2 : Fcn  Expr=u^(2/3)
  Fcn3 : Fcn  Expr=(u+1E-4)^(-3/4)
  Fcn4 : Fcn  Expr=u^0.45
  Gain1 : Gain  Gain=172  SaturateOnIntegerOverflow=on  OutDataTypeStr=Inherit: Same as input  ParamDataTypeStr=Inherit: Same as input
  Gain2 : Gain  Gain=1/10  SaturateOnIntegerOverflow=on  OutDataTypeStr=Inherit: Same as input  ParamDataTypeStr=Inherit: Same as input
  Gain3 : Gain  Gain=1/10  SaturateOnIntegerOverflow=on  OutDataTypeStr=Inherit: Same as input  ParamDataTypeStr=Inherit: Same as input
  Gain4 : Gain  Gain=320  SaturateOnIntegerOverflow=on  OutDataTypeStr=Inherit: Same as input  ParamDataTypeStr=Inherit: Same as input
  Math Function3 : Math  Operator=magnitude^2  SignedPower=on
  Math Function4 : Math  Operator=pow  SignedPower=on
  Math Function5 : Math  Operator=pow  SignedPower=on
  Product3 : Product  Inputs=3  SaturateOnIntegerOverflow=on  OutDataTypeStr=Inherit: Same as first input
  Product4 : Product  Inputs=/**  SaturateOnIntegerOverflow=on  OutDataTypeStr=Inherit: Same as first input
  Sum1 : Sum  Inputs=++|  SaturateOnIntegerOverflow=on
  n (NORSOK parameter) : Constant  Value=0.468
  z (height) : Constant  Value=Par_Wind_z
  S : Outport
  wires:
  Freqs/1 -> Gain1/1
  Gain1/1 -> Product3/1
  z (height)/1 -> Gain2/1
  Gain2/1 -> Fcn2/1, Fcn4/1
  Fcn2/1 -> Product3/2
  u10/1 -> Gain3/1
  Gain3/1 -> Fcn3/1, Math Function3/1
  Fcn3/1 -> Product3/3
  Product3/1 -> Math Function4/1  "x"
  n (NORSOK parameter)/1 -> Math Function4/2
  Math Function4/1 -> Sum1/2
  Constant2/1 -> Sum1/1
  Sum1/1 -> Math Function5/1
  Math Function5/1 -> Product4/1
  Fcn4/1 -> Gain4/1
  Math Function3/1 -> Product4/3
  Gain4/1 -> Product4/2
  Product4/1 -> S/1
  5/(3n) (NORSOK parameter)/1 -> Math Function5/2

== system demoS175WindCurrentAutopilot/Wind /Wind gust/Phase generator ==
  Trigger : TriggerPort  VariantControl=(inherit)
  Random Number : RandomNumber  Variance=3  Seed=Par_Wind_phase_seed*[1:Par_Wind_nfreq]
  "[-inf inf] to [-pi pi] " : mssSimulink/Utilities/Math Operations/[-inf inf] to [-pi pi]
  Phase : Outport
  wires:
  Random Number/1 -> "[-inf inf] to [-pi pi] "/1
  "[-inf inf] to [-pi pi] "/1 -> Phase/1
